simulink model "plasmaless_timestep"  (R2022a)
settings: Solver=FixedStepAuto  StartTime=0.0  StopTime=10.0  RelTol=1e-3
values from neighbouring files (symbols this model uses):
  A = sysd_plasmaless.A    [configure_plasmaless_model.m]    (also in timeseries_plasmaless_model.m = 10)
  B = sysd_plasmaless.B    [configure_plasmaless_model.m]
  C = sysd_plasmaless.C    [configure_plasmaless_model.m]
  D = sysd_plasmaless.D    [configure_plasmaless_model.m]
  x0 = zeros(size(A,1),1)    [run_plasmaless_model.m]
settings Model: Creator=pesamof  LastModifiedBy=pesamof

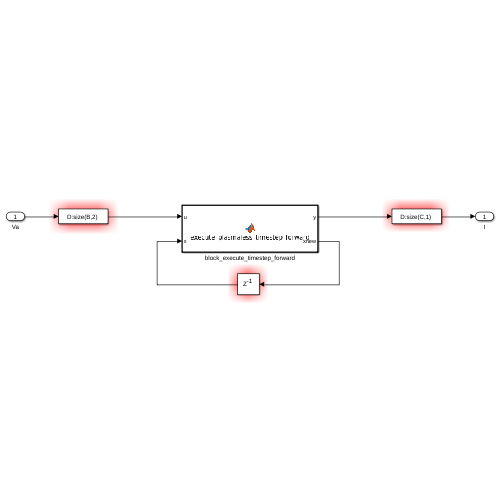
[thumbnail: Simulink's stored preview of the top-level diagram]
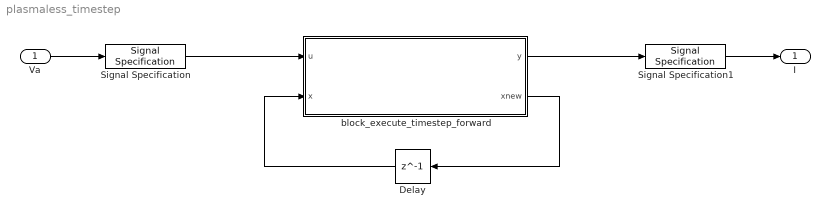
== system plasmaless_timestep ==
  Va : Inport
  Delay : Delay  DelayLength=1  InitialCondition=x0
  Signal Specification : SignalSpecification  Dimensions=size(B,2)
  Signal Specification1 : SignalSpecification  Dimensions=size(C,1)
  block_execute_timestep_forward : MATLAB Function  TreatAsAtomicUnit=on
  I : Outport
  wires:
  block_execute_timestep_forward/2(xnew) -> Delay/1
  Delay/1 -> block_execute_timestep_forward/2(x)
  block_execute_timestep_forward/1(y) -> Signal Specification1/1
  Va/1 -> Signal Specification/1
  Signal Specification/1 -> block_execute_timestep_forward/1(u)
  Signal Specification1/1 -> I/1

== matlab function plasmaless_timestep/block_execute_timestep_forward ==
  data: u input; y output; x input; xnew output; A parameter; B parameter; C parameter; D parameter
function [y,xnew] = execute_plasmaless_timestep_forward(u,x,A,B,C,D)
% run the matlab function for a forward step of the plasmaless model

[y,xnew] = plasmaless_timestep_forward(u,x,A,B,C,D);
